simulink model "mixr1_v2_dev"  (R2026a)
settings: Solver=FixedStepAuto  StopTime=inf  FixedStep=0.05  EnableMultiTasking=on
undefined symbols (not defined in the file or in its folder): mixr1_bench, student_band, student_mode, student_pumpV, student_sp
(part 2 of 2)

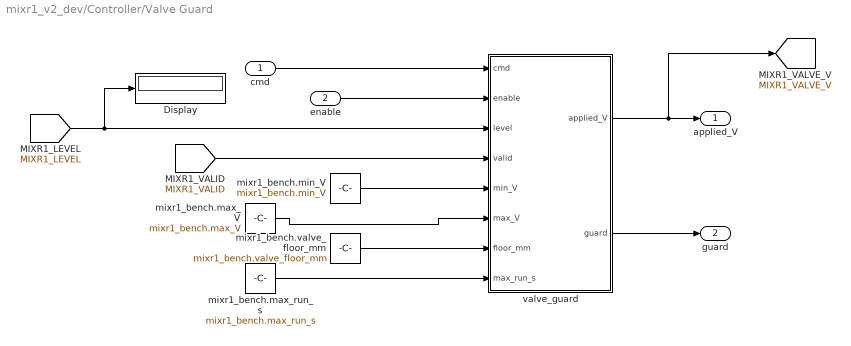
== system mixr1_v2_dev/Controller/Valve Guard ==
  cmd : Inport
  enable : Inport  Port=2
  Display : Display
  mixr1_bench.max_V : Constant  Value=mixr1_bench.max_V
  mixr1_bench.max_run_s : Constant  Value=mixr1_bench.max_run_s
  mixr1_bench.min_V : Constant  Value=mixr1_bench.min_V
  mixr1_bench.valve_floor_mm : Constant  Value=mixr1_bench.valve_floor_mm
  valve_guard : MATLAB Function  TreatAsAtomicUnit=on
  applied_V : Outport
  guard : Outport  Port=2
  tag scope: MIXR1_VALVE_V=global
  wires:
  mixr1_bench.min_V/1 -> valve_guard/5(min_V)
  mixr1_bench.max_V/1 -> valve_guard/6(max_V)
  mixr1_bench.max_run_s/1 -> valve_guard/8(max_run_s)
  mixr1_bench.valve_floor_mm/1 -> valve_guard/7(floor_mm)
  [MIXR1_LEVEL] -> Display/1, valve_guard/3(level)
  [MIXR1_VALID] -> valve_guard/4(valid)
  cmd/1 -> valve_guard/1(cmd)
  enable/1 -> valve_guard/2(enable)
  valve_guard/1(applied_V) -> [MIXR1_VALVE_V], applied_V/1
  valve_guard/2(guard) -> guard/1

== matlab function mixr1_v2_dev/Actuators/MATLAB Function ==
  data: pump_V input; valve_V input; pump_counts input; valve_counts input
function actuators(pump_V, valve_V, pump_counts, valve_counts) %#codegen
% Drives the pump and valve through act2_wrapper.c. Pi build only; PC simulation does nothing here.
% pump_V and valve_V are the guards' applied_V (read from the hidden tags MIXR1_PUMP_V and
% MIXR1_VALVE_V, so nothing but a guard can switch a device). 0 means off, anything above 0 means on.
% pump_counts and valve_counts come from the bench file and are the maximum drive for each device.
% Pump: pump_V (multimeter volts) is mapped to counts by a measured table, so pumpV now changes the PWM. Valve: fixed at valve_counts
% (on/off only). The counts-to-volts relation at the driver is still unmeasured with a scope.
coder.extrinsic('which', 'fileparts');
persistent started
if isempty(started), started = false; end
if ~coder.target('Sfun')
    srcDir = coder.const(fileparts(which('act2_wrapper.c')));
    coder.cinclude('act2_wrapper.h');
    coder.updateBuildInfo('addIncludePaths', srcDir);
    coder.updateBuildInfo('addSourcePaths',  srcDir);
    coder.updateBuildInfo('addSourceFiles', 'act2_wrapper.c');
    coder.updateBuildInfo('addLinkFlags', '-lwiringPi');
    if ~started
        coder.ceval('act2_init');
        started = true;
    end
    % Pump: pump_V is the target in volts as read by a multimeter at the pump terminals. The table below is the
    % bench calibration (24 V supply). Counts are interpolated from it and never exceed pump_counts.
    % The last point (167 counts, 12.0 V) is extrapolated from the trend, NOT measured: check it with the meter.
    CAL_V = [0 1.92 3.2 4.1 4.9 5.7 6.5 7.2 7.9 8.7 9.4 10.2 10.9 12.0];
    CAL_C = [0 12 25 37 50 62 75 87 99 112 124 137 149 167];
    t  = double(pump_V);
    pc = CAL_C(end);
    if t < CAL_V(end)
        for k = 2:numel(CAL_V)
            if t <= CAL_V(k)
                pc = CAL_C(k-1) + (CAL_C(k) - CAL_C(k-1)) * (t - CAL_V(k-1)) / (CAL_V(k) - CAL_V(k-1));
                break
            end
        end
    end
    pc = min(pc, double(pump_counts));
    if pump_V > 0, pc = max(pc, 1); end
    coder.ceval('act2_pump',  uint8(pump_V  > 0), uint16(round(pc)));
    coder.ceval('act2_valve', uint8(valve_V > 0), uint16(valve_counts));
end
end

== matlab function mixr1_v2_dev/TOF Read/level_calc ==
  data: dist input; level output; status input; newData input; gain input; intercept input; zero input; thickness input; lgain input; valid output; newOut output; raw output; corr output
function [level, valid, newOut, raw, corr] = level_calc(dist, status, newData, gain, intercept, zero, thickness, lgain) %#codegen
% Replaces tof_correct and the level maths that used to sit inside fluid_ctrl.
%   corr  = (raw - intercept) / gain          same formula as tof_correct
%   level = max(0, lgain * (zero - median3(corr) - thickness))   same as fluid_ctrl v1
% valid is true only if a good frame (status 0, corr in 30..2000 mm) arrived within the
% last MAX_AGE steps. Bad or missing frames never refresh it, so valid drops after 0.6 s.
% 12 steps = 3 frame periods at the longest allowed budget (200 ms), so 2 lost frames are tolerated.
MAX_AGE = 12;

persistent buf n age have lvl rawV corrV
if isempty(buf)
    buf = zeros(1,3); n = 0; age = 1e6; have = false;
    lvl = 0; rawV = 0; corrV = 0;
end

newOut = (newData == 1);
if newData == 1
    d = (double(dist) - intercept) / gain;
    if status == 0 && d > 30 && d <= 2000
        if age > MAX_AGE, n = 0; end              % first good frame after a dropout: forget old readings
        buf  = [buf(2:3), d];
        n    = min(n + 1, 3);
        age  = 0;
        have = true;
        rawV = double(dist);
        corrV = d;
        lvl  = max(0, lgain * (zero - median(buf(4-n:3)) - thickness));
    else
        age = min(age + 1, 1e6);
    end
else
    age = min(age + 1, 1e6);
end

level = lvl;
valid = have && (age <= MAX_AGE);
raw   = rawV;
corr  = corrV;
end

== matlab function mixr1_v2_dev/TOF Read/tof_read ==
  data: offset_mm input; dist output; budget_ms input; status output; newData output
function [dist, status, newData] = tof_read(offset_mm, budget_ms) %#codegen
% Level Sensor driver. Real VL53L4CD on the Pi, simulated frames in PC simulation.
% offset_mm and budget_ms come from the bench file through Constant blocks.
coder.extrinsic('which', 'fileparts');
dist    = uint16(0);
status  = uint8(255);
newData = uint8(0);

persistent k frame lastDist started
if isempty(k)
    k = uint32(0);
    frame = uint32(0);
    lastDist = uint16(0);
    started = false;
end

if coder.target('Sfun')
    % PC simulation only: a frame every 4th step (5 Hz). Raw distance sweeps 398..202 mm
    % (level about 8..202 mm with the default bench). Steps 400..519 are a dropout,
    % so the stale-data logic can be seen working.
    k = k + uint32(1);
    stall = (k >= uint32(400)) && (k < uint32(520));
    if mod(k, uint32(4)) == 0 && ~stall
        frame = frame + uint32(1);
        lastDist = uint16(400) - uint16(2) * uint16(mod(frame, uint32(100)));
        newData = uint8(1);
    end
    dist = lastDist;
    if frame > 0
        status = uint8(0);
    end
else
    srcDir = coder.const(fileparts(which('tof_wrapper.c')));
    coder.cinclude('tof_wrapper.h');
    coder.updateBuildInfo('addIncludePaths', srcDir);
    coder.updateBuildInfo('addSourcePaths',  srcDir);
    coder.updateBuildInfo('addSourceFiles', 'tof_wrapper.c');
    coder.updateBuildInfo('addSourceFiles', 'VL53L4CD_api.c');
    coder.updateBuildInfo('addSourceFiles', 'platform.c');

    if ~started
        coder.ceval('tof_init', int16(offset_mm), uint16(budget_ms));
        started = true;
    end
    coder.ceval('tof_step', coder.wref(dist), coder.wref(status), coder.wref(newData));
end
end

== matlab function mixr1_v2_dev/Controller/Controller/MATLAB Function ==
  data: mode input; pump_V output; setpoint input; band_pct input; pumpV input; valveV input; level input; valid input; min_V input; max_V input; min_band input; floor_mm input; max_level input; margin input; pump_en output; valve_V output; valve_en output; status output; sp_used output; band_used output
function [pump_V, pump_en, valve_V, valve_en, status, sp_used, band_used] = controller( ...
        mode, setpoint, band_pct, pumpV, valveV, level, valid, ...
        min_V, max_V, min_band, floor_mm, max_level, margin) %#codegen
% MIXR1 Controller (locked block). Students set only: mode, setpoint, band_pct (and pumpV where it is exposed).
% band_pct: half-width of the switching window as a percentage of the setpoint in use (students use 5 to 10).
% valveV is not a student knob: the valve is on or off, so valveV is fixed at 6 V (the Constant stays at 6).
% mode 0: off
% mode 1: pump always on at pumpV, the valve switches (opens above setpoint+band, closes below setpoint-band)
% mode 2: valve always open at valveV, the pump switches (on below setpoint-band, off above setpoint+band)
% mode 3: instructor drain. Valve open, pump off. The Valve Guard closes the valve at the 2 mm floor. Not a student mode.
% The last six inputs come from the bench file (Constant blocks inside this block), not from students.
% status: 0 off | 1 raising | 2 lowering | 3 no valid level | 4 waiting for mode 0 after start
% Startup lockout: on the Pi nothing runs until mode has been 0 at least once since the program started,
% so a model that starts with mode 1 or 2 left on cannot switch the pump or valve by itself.
% In Simulink PC simulation (the Sfun target) the lockout is skipped.
persistent sw prevMode armed
if isempty(sw), sw = false; prevMode = 0; armed = coder.target('Sfun'); end   % sw = the switching device is on

trip      = max_level - margin;                              % the Pump guard cuts at this level
p         = min(max(band_pct, 0), 50) / 100;                 % percent -> fraction
sp1       = min(setpoint, trip / (1 + p));                   % top of the window never above the trip level
band_used = min(max(sp1 * p, min_band), (trip - floor_mm) / 2);
sp_used   = min(max(sp1, floor_mm + band_used), trip - band_used);
pump_V    = min(max(pumpV,  min_V), max_V);                  % volts at the load, min_V..max_V
valve_V   = min(max(valveV, min_V), max_V);

if mode ~= prevMode, sw = false; end                         % changing mode restarts the switching
prevMode = mode;

if mode == 0, armed = true; end
wanted  = (mode == 1 || mode == 2 || mode == 3);
active  = armed && wanted;
pump_en = false;
valve_en = false;
status  = uint8(0);

if ~active || ~valid
    sw = false;
    if active
        status = uint8(3);                                   % wanted to run, but no valid level
    elseif wanted
        status = uint8(4);                                   % mode is on but the controller is not armed yet
    end
elseif mode == 3
    sw       = false;
    pump_en  = false;
    valve_en = true;
    status   = uint8(2);                                     % lowering
elseif mode == 1
    if level >= sp_used + band_used
        sw = true;
    elseif level <= sp_used - band_used
        sw = false;
    end
    pump_en  = true;
    valve_en = sw;
    status   = uint8(1 + double(sw));                        % valve open: lowering
else
    if level <= sp_used - band_used
        sw = true;
    elseif level >= sp_used + band_used
        sw = false;
    end
    pump_en  = sw;
    valve_en = true;
    status   = uint8(2 - double(sw));                        % pump on: raising
end
end

== matlab function mixr1_v2_dev/Controller/Pump Guard/pump_guard ==
  data: cmd input; applied_V output; enable input; level input; valid input; min_V input; max_V input; trip input; max_run_s input; guard output
function [applied_V, guard] = pump_guard(cmd, enable, level, valid, min_V, max_V, trip, max_run_s) %#codegen
% Pump safety guard (locked block). Forces the pump off whatever the Controller or a student asks.
% cmd, enable : from the Controller or a Dashboard switch (volts at the load, on/off)
% level, valid: from the Level Sensor
% min_V, max_V, trip, max_run_s: bench file (Constant blocks inside this block)
%   trip = max_level_mm - ceiling_margin_mm
% guard: 0 ok | 1 no valid level | 3 level at the ceiling | 4 continuous-run limit
DT = 0.05;  RELEASE = 5;  REST_S = 2;
persistent atCeiling runSteps offSteps latched
if isempty(atCeiling)
    atCeiling = false; runSteps = 0; offSteps = 0; latched = false;
end

want  = enable && cmd > 0;                       % NaN or negative commands mean off
sees  = valid && isfinite(level);

if sees
    if level >= trip
        atCeiling = true;
    elseif level <= trip - RELEASE               % resumes only 5 mm below the trip level
        atCeiling = false;
    end
end

if want                                          % run limit is cleared after REST_S seconds commanded off
    offSteps = 0;
else
    offSteps = min(offSteps + 1, 1e6);
    if offSteps * DT >= REST_S
        runSteps = 0;
        latched  = false;
    end
end

if ~sees
    guard = uint8(1);
elseif atCeiling
    guard = uint8(3);
elseif latched
    guard = uint8(4);
else
    guard = uint8(0);
end

if want && guard == 0
    runSteps = runSteps + 1;
    if runSteps * DT >= max_run_s
        latched = true;
        guard   = uint8(4);
    end
end

applied_V = 0;
if want && guard == 0
    applied_V = min(max(cmd, min_V), max_V);
end
end

== matlab function mixr1_v2_dev/Controller/Valve Guard/valve_guard ==
  data: cmd input; applied_V output; enable input; level input; valid input; min_V input; max_V input; floor_mm input; max_run_s input; guard output
function [applied_V, guard] = valve_guard(cmd, enable, level, valid, min_V, max_V, floor_mm, max_run_s) %#codegen
% Valve safety guard (locked block). Forces the valve closed whatever the Controller or a student asks.
% cmd, enable : from the Controller or a Dashboard switch (volts at the load, on/off)
% level, valid: from the Level Sensor
% min_V, max_V, floor_mm, max_run_s: bench file (Constant blocks inside this block)
% guard: 0 ok | 1 no valid level | 4 continuous-open limit | 5 level at the floor (valve held closed)
DT = 0.05;  RELEASE = 2;  REST_S = 2;
persistent atFloor runSteps offSteps latched
if isempty(atFloor)
    atFloor = false; runSteps = 0; offSteps = 0; latched = false;
end

want = enable && cmd > 0;                        % NaN or negative commands mean closed
sees = valid && isfinite(level);

if sees
    if level <= floor_mm
        atFloor = true;
    elseif level >= floor_mm + RELEASE           % reopens only 2 mm above the floor
        atFloor = false;
    end
end

if want                                          % run limit is cleared after REST_S seconds commanded closed
    offSteps = 0;
else
    offSteps = min(offSteps + 1, 1e6);
    if offSteps * DT >= REST_S
        runSteps = 0;
        latched  = false;
    end
end

if ~sees
    guard = uint8(1);
elseif atFloor
    guard = uint8(5);
elseif latched
    guard = uint8(4);
else
    guard = uint8(0);
end

if want && guard == 0
    runSteps = runSteps + 1;
    if runSteps * DT >= max_run_s
        latched = true;
        guard   = uint8(4);
    end
end

applied_V = 0;
if want && guard == 0
    applied_V = min(max(cmd, min_V), max_V);
end
end
